simulink subsystem "DcmFromAxis"  (R2024b)
settings: Solver=VariableStepAuto  StartTime=0.0  StopTime=10.0  RelTol=1e-3
settings Model: Creator=marco  LastModifiedBy=ferru

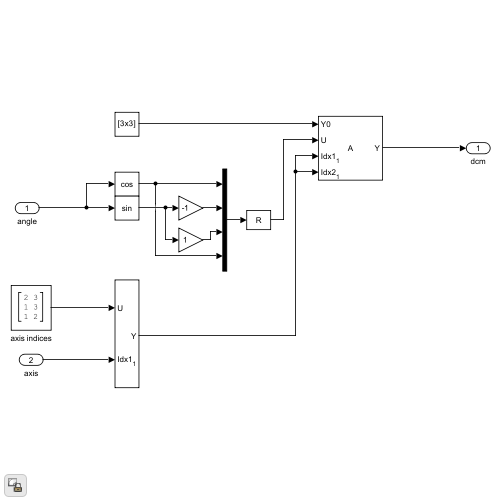
[thumbnail: Simulink's stored preview of the top-level diagram]
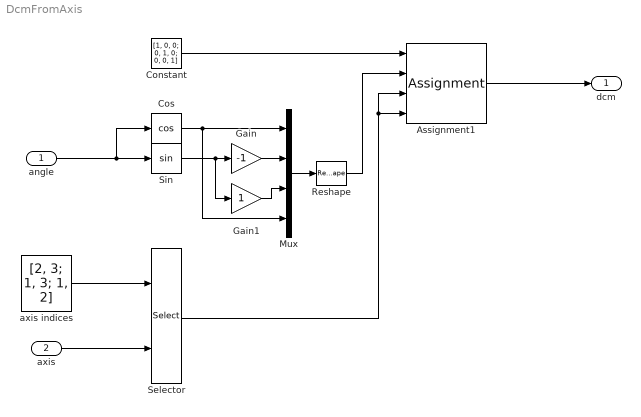
== system DcmFromAxis ==
  angle : Inport
  axis : Inport  Port=2  OutMin=1  OutMax=3
  Assignment1 : Assignment  NumberOfDimensions=2  DiagnosticForDimensions=Warning  IndexOptions=Index vector (port),Index vector (port)  Indices=1:2,1:2  OutputSizes=1,1
  Constant : Constant  Value=[1, 0, 0; 0, 1, 0; 0, 0, 1]  VectorParams1D=off
  Cos : Trigonometry  Operator=cos
  Gain : Gain  Gain=-1
  Gain1 : Gain
  Mux : Mux
  Reshape : Reshape  OutputDimensionality=Customize  OutputDimensions=[2, 2]
  Selector : Selector  NumberOfDimensions=2  InputPortWidth=3  IndexOptions=Index vector (port),Select all  Indices=[1 3],1  OutputSizes=1,1
  Sin : Trigonometry
  axis indices : Constant  Value=[2, 3; 1, 3; 1, 2]
  dcm : Outport
  wires:
  angle/1 -> Sin/1, Cos/1
  Constant/1 -> Assignment1/1
  Cos/1 -> Mux/4, Mux/1
  Sin/1 -> Gain/1, Gain1/1
  Mux/1 -> Reshape/1
  axis/1 -> Selector/2
  axis indices/1 -> Selector/1
  Selector/1 -> Assignment1/4, Assignment1/3
  Assignment1/1 -> dcm/1
  Reshape/1 -> Assignment1/2
  Gain1/1 -> Mux/3
  Gain/1 -> Mux/2
